simulink model "DCServomotorWResLoad_PID_Quanser"  (R2024b)
settings: Solver=VariableStepAuto  StartTime=0.0  StopTime=5  MaxStep=0.00001  MinStep=3e-09  RelTol=1e-1
undefined symbols (not defined in the file): Kd, Ki, Kp, Kw, sens, TL
settings Model: Creator=liliy  LastModifiedBy=lenovo
settings SolverCC: ZeroCrossAlgorithm=Adaptive
settings DataIOCC: ReturnWorkspaceOutputs=off
settings DebuggingCC: IgnoredZcDiagnostic=none

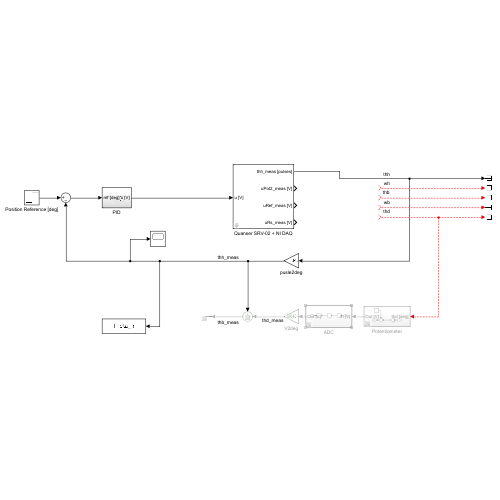
[thumbnail: Simulink's stored preview of the top-level diagram]
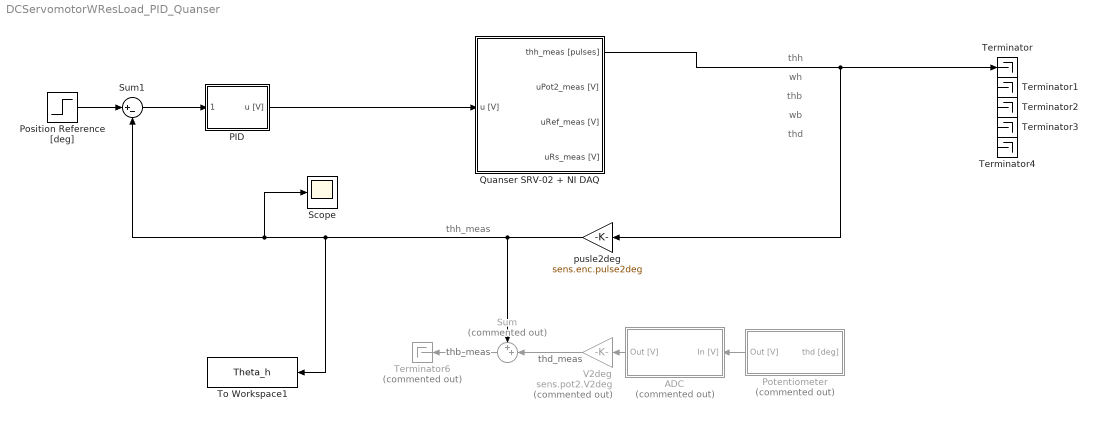
== system DCServomotorWResLoad_PID_Quanser ==
  note: thd
  note: wb
  note: thb
  note: wh
  note: thh
  note: thh_meas
  note: thd_meas
  note: thb_meas
  ADC : Subsystem  Commented=on
  PID : Subsystem
  Position Reference [deg] : Step  After=50  SampleTime=0
  Potentiometer : Subsystem  Commented=on
  Quanser SRV-02 + NI DAQ : Subsystem  mask(Quanser SRV-02 (with resonant load) + NI DAQ){Ts=0.001, fricType=Coulomb + viscous, lockShaft=off, beamInitPos=10}
      mask prompts: Ts "NI DAQ Sample Time:"; fricType "Friction model"; lockShaft "Lock motor shaft"; beamInitPos "Beam initial position [deg]:"
      mask help: Quanser SRV-02 (with resonant load) + NI DAQ model.
      mask init:
      | %%
      | % Riccardo Antonello (riccardo.antonello@unipd.it)
      | %
      | % April 28, 2020
      | %
      | % Dept. of Information Engineering, University of Padova
      | %
      | 
      | %%  Conversion gains
      | deg2rad = pi/180;                   %   [deg]   -> [rad]
      | rad2deg = 180/pi;                   %   [rad]   -> [deg]
      | 
      | 
      | %%  Sensors data
      | 
      | %   shunt resistor
      | sens.curr.Rs = 0.5;   
      | 
      | %   Hewlett-Packard HEDS-5540#A06 optical encoder
      | sens.enc.ppr = 500*4;                                                   %   pulses per rotation
      | sens.enc.pulse2deg = 360/sens.enc.ppr;                                  %   [pulses] -> [deg]
      | sens.enc.pulse2rad = 2*pi/sens.enc.ppr;                                 %   [pulses] -> [rad]
      | sens.enc.deg2pulse = sens.enc.ppr/360;                                  %   [deg] -> [pulses]
      | sens.enc.rad2pulse = sens.enc.ppr/2/pi;                                 %   [rad] -> [pulses]
      | 
      | %   potentiometer 2 (Spectrol 357-0-0-103) - installed on hub
      | sens.pot2.range.R      = 10e3;                                          %   ohmic value range 
      | sens.pot2.range.V      = 5;                                             %   voltage range
      | sens.pot2.range.th_deg = 340;                                           %   angle range [deg]
      | sens.pot2.range.th     = sens.pot2.range.th_deg * deg2rad;              %   angle range [rad]                           
      | sens.pot2.deg2V        = sens.pot2.range.V / sens.pot2.range.th_deg;    %   sensitivity [V/deg]
      | sens.pot2.rad2V        = sens.pot2.range.V / sens.pot2.range.th;        %   sensitivity [V/rad]
      | sens.pot2.V2deg        = 1/sens.pot2.deg2V;                             %   conversion gain [V] -> [deg]
      | sens.pot2.V2rad        = 1/sens.pot2.rad2V;                             %   conversion gain [V] -> [rad]
      | sens.pot2.noise.var    = 3.5e-7;                                        %   out noise variance [V^2]
      | 
      | 
      | %%  Data acquisition board (daq) data
      | 
      | %   NI PCI-6221 DAC data
      | daq.dac.bits = 16;                                  %   resolution (bits)
      | daq.dac.fs   = 10;                                  %   full scale 
      | daq.dac.q    = 2*daq.dac.fs/(2^daq.dac.bits-1);     %	quantization
      | 
      | %   NI PCI-6221 ADC data
      | daq.adc.bits = 16;                                  %   resolution (bits)
      | daq.adc.fs   = 10;                                  %   full scale (as set in SLDRT Analog Input block)
      | daq.adc.q    = 2*daq.adc.fs/(2^daq.adc.bits-1);     %   quantization   
      | 
      | 
      | %%  Set beam initial position
      | % SRV02Handle = find_system(gcb, ...
      | %     'LookUnderMasks', 'on', ...
      | %     'FindAll', 'on', ...
      | %     'FollowLinks', 'on', ...
      | %     'SearchDepth', '1', ...
      | %     'BlockType', 'ModelReference', ...
      | %     'Name', 'Quanser SRV-02');
      | %
      | % %get_param(SRV02Handle, 'InstanceParameters')
      | % InstanceParams = get_param(SRV02Handle, 'InstanceParameters');
      | % for k = 1:length(InstanceParams)
      | %     if strcmp(InstanceParams(k).Name, 'thb0')
      | %         if lockShaft
      | %             InstanceParams(k).Value = sprintf('%f', beamInitPos);
      | %         else
      | %             InstanceParams(k).Value = sprintf('%f', 0);    
      | %         end
      | %         set_param(SRV02Handle, 'InstanceParameters', InstanceParams);
      | %         break;
      | %     end
      | % end
      | 
      | if lockShaft
      |     thb0 = beamInitPos;
      | else
      |     thb0 = 0;    
      | end
      | 
      | 
      | %%  Mask initialization
      | if lockShaft
      |     
      |     %   find Inport handle
      |     InPortHandle = find_system(gcb, ...
      |         'LookUnderMasks', 'on', ...
      |         'FindAll', 'on', ...
      |         'FollowLinks', 'on', ...
      |         'SearchDepth', '1', ...
      |         'BlockType', 'Inport', ...
      |         'Name', 'u [V]');
      |     
      |     if ~isempty(InPortHandle)
      |     
      |         %   find DAC handle
      |         DACHandle = find_system(gcb, ...
      |             'LookUnderMasks', 'on', ...
      |             'FindAll', 'on', ...
      |             'FollowLinks', 'on', ...
      |             'SearchDepth', '1', ...
      |             'BlockType', 'SubSystem', ...
      |             'Name', 'DAC');  
      | 
      |         %   remove Inport output connection   
      |         InportConn = get_param(InPortHandle, 'PortConnectivity');
      |         delete_line(gcb, InportConn.Position);
      | 
      |         %   remove Inport block
      |         delete_block(InPortHandle);
      | 
      |         %   add Constant block
      |         ConstantHandle = add_block( ...
      |             'simulink/Sources/Constant', [gcb, '/u [V]'], ...
      |             'Position', [20   -37    50   -23], ...
      |             'Value', '0');
      | 
      |         %   connect Constant to DAC block
      |         DACPortHandles = get_param(DACHandle, 'PortHandles');
      |         ConstantPortHandles = get_param(ConstantHandle, 'PortHandles');
      |         add_line(gcb, ConstantPortHandles.Outport(1), DACPortHandles.Inport(1));
      |     
      |     end
      |     
      | else
      |     
      |     %   find Constant handle
      |     ConstantHandle = find_system(gcb, ...
      |         'LookUnderMasks', 'on', ...
      |         'FindAll', 'on', ...
      |         'FollowLinks', 'on', ...
      |         'SearchDepth', '1', ...
      |         'BlockType', 'Constant', ...
      |         'Name', 'u [V]');
      |     
      |     if ~isempty(ConstantHandle)
      |     
      |         %   find DAC handle
      |         DACHandle = find_system(gcb, ...
      |             'LookUnderMasks', 'on', ...
      |             'FindAll', 'on', ...
      |             'FollowLinks', 'on', ...
      |             'SearchDepth', '1', ...
      |             'BlockType', 'SubSystem', ...
      |             'Name', 'DAC');  
      |  
      |         %   remove Constant output connection   
      |         ConstantConn = get_param(ConstantHandle, 'PortConnectivity');
      |         delete_line(gcb, ConstantConn.Position);
      | 
      |         %   remove Inport block
      |         delete_block(ConstantHandle);   
      | 
      |         %   add Inport block
      |         InportHandle = add_block( ...
      |             'simulink/Sources/In1', [gcb, '/u [V]'], ...
      |             'Position', [20   -37    50   -23], ...
      |             'Port', '1');
      | 
      |         %   connect Constant to DAC block
      |         DACPortHandles = get_param(DACHandle, 'PortHandles');
      |         InportPortHandles = get_param(InportHandle, 'PortHandles');
      |         add_line(gcb, InportPortHandles.Outport(1), DACPortHandles.Inport(1));
      |     
      |      end
      |     
      | end
      mask Help:
      | Riccardo Antonello (antonello@dei.unipd.it)
      | 
      | April 28, 2020
      | 
      | Dept. of Information Engineering, University of Padova
      mask TypeOptions fricType: Coulomb + viscous | Karnopp
      mask Callback lockShaft:
      | %   get status of check box
      | lockShaft = get_param(gcb, 'lockShaft');
      | 
      | %   get current value of MaskVisibilities property
      | maskVisibilities = get_param(gcb, 'MaskVisibilities');
      | 
      | %   set visibility of the dialog box element
      | if strcmp(lockShaft, 'on')
      |     maskVisibilities{4} = 'on';
      | else
      |     maskVisibilities{4} = 'off';
      | end
      | 
      | % Set the 'MaskVisibilities' property for each parameter in mask
      | set_param( gcb, 'MaskVisibilities', maskVisibilities);
  Scope : Scope
  Sum : Sum  Commented=on  Inputs=++|
  Sum1 : Sum  Inputs=|+-
  Terminator{,1..4} (5 alike) : Terminator
  Terminator6 : Terminator  Commented=on
  To Workspace1 : ToWorkspace  VariableName=Theta_h  SaveFormat=Structure With Time  SampleTime=0.001
  V2deg : Gain  Commented=on  Gain=sens.pot2.V2deg
  pusle2deg : Gain  Gain=sens.enc.pulse2deg
  wires:
  ? -> Terminator1/1
  ? -> Terminator2/1
  ? -> Terminator3/1
  ? -> Potentiometer/1(thd [deg]), Terminator4/1
  Quanser SRV-02 + NI DAQ/1(thh_meas [pulses]) -> pusle2deg/1, Terminator/1
  pusle2deg/1 -> To Workspace1/1, Scope/1, Sum1/2, Sum/1
  Potentiometer/1(Out [V]) -> ADC/1(In [V])
  ADC/1(Out [V]) -> V2deg/1
  Sum/1 -> Terminator6/1
  V2deg/1 -> Sum/2
  Position Reference [deg]/1 -> Sum1/1
  Sum1/1 -> PID/1(ref [deg])
  PID/1(u [V]) -> Quanser SRV-02 + NI DAQ/1(u [V])

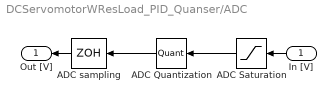
== system DCServomotorWResLoad_PID_Quanser/ADC ==
  In [V] : Inport
  ADC Quantization : Quantizer  QuantizationInterval=daq.adc.q
  ADC Saturation : Saturate  UpperLimit=10  LowerLimit=10
  ADC sampling : ZeroOrderHold  SampleTime=1e-03
  Out [V] : Outport
  wires:
  ADC sampling/1 -> Out [V]/1
  ADC Saturation/1 -> ADC Quantization/1
  ADC Quantization/1 -> ADC sampling/1
  In [V]/1 -> ADC Saturation/1

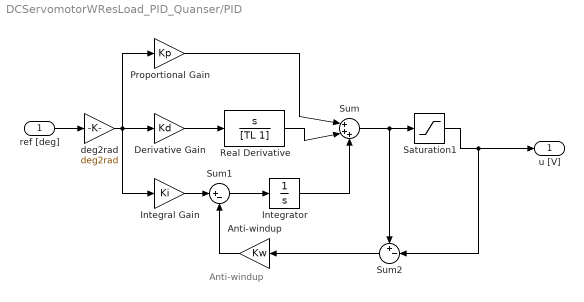
== system DCServomotorWResLoad_PID_Quanser/PID ==
  note: Anti-windup
  ref [deg] : Inport
  Anti-windup : Gain  Gain=Kw
  Derivative Gain : Gain  Gain=Kd
  Integral Gain : Gain  Gain=Ki
  Integrator : Integrator
  Proportional Gain : Gain  Gain=Kp
  Real Derivative : TransferFcn  Numerator=[1 0]  Denominator=[TL 1]
  Saturation1 : Saturate  UpperLimit=12  LowerLimit=-12
  Sum : Sum  Inputs=|+++
  Sum1 : Sum  Inputs=|+-
  Sum2 : Sum  Inputs=+-|
  deg2rad : Gain  Gain=deg2rad
  u [V] : Outport
  wires:
  Integrator/1 -> Sum/3
  Real Derivative/1 -> Sum/2
  Derivative Gain/1 -> Real Derivative/1
  Proportional Gain/1 -> Sum/1
  ref [deg]/1 -> deg2rad/1
  deg2rad/1 -> Proportional Gain/1, Integral Gain/1, Derivative Gain/1
  Sum/1 -> Saturation1/1, Sum2/1
  Saturation1/1 -> Sum2/2, u [V]/1
  Integral Gain/1 -> Sum1/1
  Anti-windup/1 -> Sum1/2
  Sum2/1 -> Anti-windup/1
  Sum1/1 -> Integrator/1

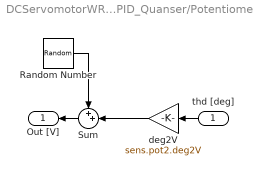
== system DCServomotorWResLoad_PID_Quanser/Potentiometer ==
  thd [deg] : Inport
  Random Number : RandomNumber  Variance=3.5*10e-07  SampleTime=1e-03
  Sum : Sum  Inputs=++|
  deg2V : Gain  Gain=sens.pot2.deg2V
  Out [V] : Outport
  wires:
  Random Number/1 -> Sum/1
  deg2V/1 -> Sum/2
  Sum/1 -> Out [V]/1
  thd [deg]/1 -> deg2V/1

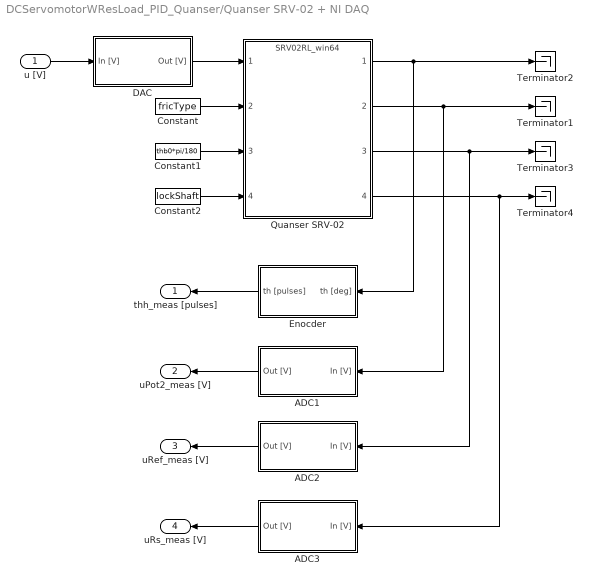
== system DCServomotorWResLoad_PID_Quanser/Quanser SRV-02 + NI DAQ ==
  u [V] : Inport
  ADC1 : Subsystem
  ADC2 : Subsystem
  ADC3 : Subsystem
  Constant : Constant  Value=fricType
  Constant1 : Constant  Value=thb0*pi/180  SampleTime=Inf
  Constant2 : Constant  Value=lockShaft  SampleTime=Inf
  DAC : Subsystem
  Enocder : Subsystem
  Quanser SRV-02 : ModelReference  ModelNameDialog=SRV02RL_win64.slxp  ModelReferenceVersion=1.76  CopyOfModelProtected=on
  Terminator{1..4} (4 alike) : Terminator
  thh_meas [pulses] : Outport
  uPot2_meas [V] : Outport  Port=2
  uRef_meas [V] : Outport  Port=3
  uRs_meas [V] : Outport  Port=4
  wires:
  Enocder/1(th [pulses]) -> thh_meas [pulses]/1
  ADC3/1(Out [V]) -> uRs_meas [V]/1
  DAC/1(Out [V]) -> Quanser SRV-02/1
  Quanser SRV-02/2 -> ADC1/1(In [V]), Terminator1/1
  Quanser SRV-02/1 -> Terminator2/1, Enocder/1(th [deg])
  Constant/1 -> Quanser SRV-02/2
  Quanser SRV-02/3 -> ADC2/1(In [V]), Terminator3/1
  ADC1/1(Out [V]) -> uPot2_meas [V]/1
  Constant1/1 -> Quanser SRV-02/3
  Constant2/1 -> Quanser SRV-02/4
  Quanser SRV-02/4 -> ADC3/1(In [V]), Terminator4/1
  ADC2/1(Out [V]) -> uRef_meas [V]/1
  u [V]/1 -> DAC/1(In [V])

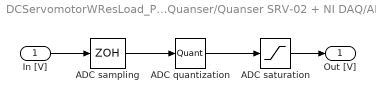
== system DCServomotorWResLoad_PID_Quanser/Quanser SRV-02 + NI DAQ/ADC1 ==
  In [V] : Inport
  ADC quantization : Quantizer  QuantizationInterval=daq.adc.q
  ADC sampling : ZeroOrderHold  SampleTime=Ts
  ADC saturation : Saturate  UpperLimit=daq.adc.fs  LowerLimit=-daq.adc.fs
  Out [V] : Outport
  wires:
  ADC saturation/1 -> Out [V]/1
  ADC sampling/1 -> ADC quantization/1
  In [V]/1 -> ADC sampling/1
  ADC quantization/1 -> ADC saturation/1

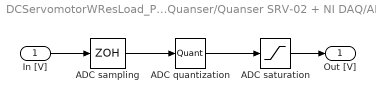
== system DCServomotorWResLoad_PID_Quanser/Quanser SRV-02 + NI DAQ/ADC2 ==
  In [V] : Inport
  ADC quantization : Quantizer  QuantizationInterval=daq.adc.q
  ADC sampling : ZeroOrderHold  SampleTime=Ts
  ADC saturation : Saturate  UpperLimit=daq.adc.fs  LowerLimit=-daq.adc.fs
  Out [V] : Outport
  wires:
  ADC quantization/1 -> ADC saturation/1
  In [V]/1 -> ADC sampling/1
  ADC sampling/1 -> ADC quantization/1
  ADC saturation/1 -> Out [V]/1

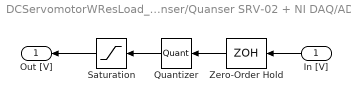
== system DCServomotorWResLoad_PID_Quanser/Quanser SRV-02 + NI DAQ/ADC3 ==
  In [V] : Inport
  Quantizer : Quantizer  QuantizationInterval=daq.adc.q
  Saturation : Saturate  UpperLimit=daq.adc.fs  LowerLimit=-daq.adc.fs
  Zero-Order Hold : ZeroOrderHold  SampleTime=Ts
  Out [V] : Outport
  wires:
  Saturation/1 -> Out [V]/1
  In [V]/1 -> Zero-Order Hold/1
  Quantizer/1 -> Saturation/1
  Zero-Order Hold/1 -> Quantizer/1

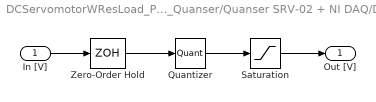
== system DCServomotorWResLoad_PID_Quanser/Quanser SRV-02 + NI DAQ/DAC ==
  In [V] : Inport
  Quantizer : Quantizer  QuantizationInterval=daq.dac.q
  Saturation : Saturate  UpperLimit=daq.dac.fs  LowerLimit=-daq.dac.fs
  Zero-Order Hold : ZeroOrderHold  SampleTime=Ts
  Out [V] : Outport
  wires:
  Quantizer/1 -> Saturation/1
  In [V]/1 -> Zero-Order Hold/1
  Zero-Order Hold/1 -> Quantizer/1
  Saturation/1 -> Out [V]/1

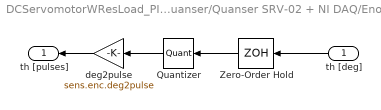
== system DCServomotorWResLoad_PID_Quanser/Quanser SRV-02 + NI DAQ/Enocder ==
  th [deg] : Inport
  Quantizer : Quantizer  QuantizationInterval=sens.enc.pulse2deg
  Zero-Order Hold : ZeroOrderHold  SampleTime=Ts
  deg2pulse : Gain  Gain=sens.enc.deg2pulse
  th [pulses] : Outport
  wires:
  Quantizer/1 -> deg2pulse/1
  th [deg]/1 -> Zero-Order Hold/1
  Zero-Order Hold/1 -> Quantizer/1
  deg2pulse/1 -> th [pulses]/1
